simulink model "radia_optuna_teaching"  (R2026a)
settings: Solver=FixedStepDiscrete  StopTime=1.4  FixedStep=0.1
PreLoadFcn:
  | radia.simulink.makeOptunaMonitorBusObject();
model workspace (MAT data in the model file):
  radia_optuna_teaching_exercise = "quadratic"
  x = 0
settings Model: Creator=Administrator  LastModifiedBy=Administrator

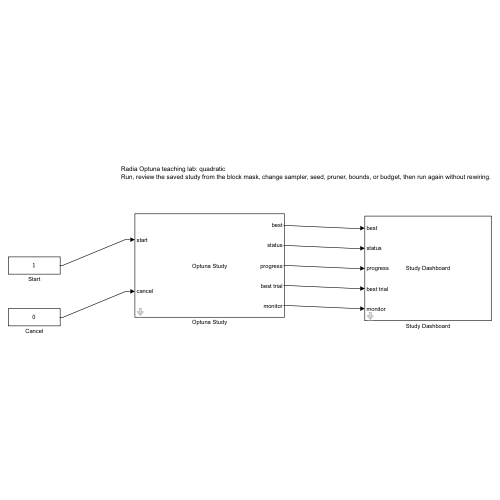
[thumbnail: Simulink's stored preview of the top-level diagram]
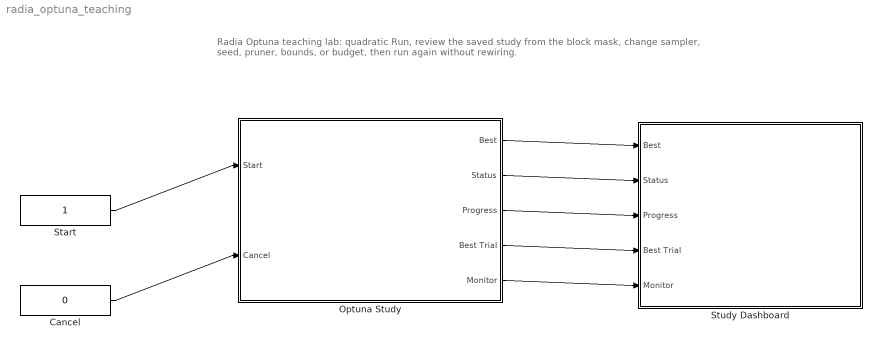
== system radia_optuna_teaching ==
  note: Radia Optuna teaching lab: quadratic
      | Run, review the saved study from the block mask, change sampler, seed, pruner, bounds, or budget, then run again without rewiring.
  Cancel : Constant  Value=0
  Optuna Study : Subsystem  mask{objective_fcn='radia.optuna.teachingQuadraticObjective', num_trials=12, directions="minimize", storage_path='C:\temp\radia_optuna_teaching_quadratic.mat', sample_time_s=0.10000000000000001, live_visualization=off, sampler_name=tpe, seed=20260829, pruner_name=median, parameter_spec=radia.optuna.OptimizationParameter('x',Value=0,Minimum=-1,Maximum=1), model_name='radia_optuna_teaching', selected_trial=-1}
      mask prompts: objective_fcn "Objective function"; num_trials "Total trial budget"; directions "Objective directions"; storage_path "Study MAT file"; sample_time_s "Trial sample time (s)"; live_visualization "External MATLAB monitor"; sampler_name "Sampler"; seed "Sampler seed ([] = fresh)"; pruner_name "Pruner"; parameter_spec "OptimizationParameter array"; model_name "Model to update"; selected_trial "Trial to apply (-1 = best)"
      mask help: Compact MATLAB-native Optuna study. Change the sampler, seed, pruner, search space, or total trial budget in this dialog and run again; the MAT study resumes without changing wiring. OptunaMonitorBusV1 exposes fixed scalar telemetry.
      mask init:
      | radia.simulink.makeOptunaMonitorBusObject();set_param([gcb '/Advanced Runtime'],'Parameters','objective_fcn,num_trials,directions,storage_path,sample_time_s,strcmp(live_visualization,''on''),struct(''Name'',sampler_name,''Seed'',seed,''Pruner'',pruner_name,''Parameters'',parameter_spec,''ModelName'',model_name)');
      mask TypeOptions sampler_name: auto | random | tpe | cmaes | motpe | nsgaii | gp | nsgaiii | bruteforce | qmc
      mask TypeOptions pruner_name: none | median | hyperband | percentile | patient | successivehalving | threshold
      mask DialogControl review_study Prompt: Review saved study
      mask DialogControl review_study Callback: radia.simulink.reviewOptunaStudy(gcb);
      mask DialogControl apply_trial Prompt: Apply selected trial
      mask DialogControl apply_trial Callback: radia.simulink.applyOptunaTrial(gcb,selected_trial);
      mask Display: disp('Optuna Study');port_label('input',1,'start');port_label('input',2,'cancel');port_label('output',1,'best');port_label('output',2,'status');port_label('output',3,'progress');port_label('output',4,'best trial');port_label('output',5,'monitor');
  Start : Constant
  Study Dashboard : Subsystem
      mask help: Compact live progress plus workspace logs. Full trial history remains in the Optuna Study MAT file.
      mask Display: disp('Study Dashboard');port_label('input',1,'best');port_label('input',2,'status');port_label('input',3,'progress');port_label('input',4,'best trial');port_label('input',5,'monitor');
  wires:
  Start/1 -> Optuna Study/1(Start)
  Cancel/1 -> Optuna Study/2(Cancel)
  Optuna Study/1(Best) -> Study Dashboard/1(Best)
  Optuna Study/2(Status) -> Study Dashboard/2(Status)
  Optuna Study/3(Progress) -> Study Dashboard/3(Progress)
  Optuna Study/4(Best Trial) -> Study Dashboard/4(Best Trial)
  Optuna Study/5(Monitor) -> Study Dashboard/5(Monitor)

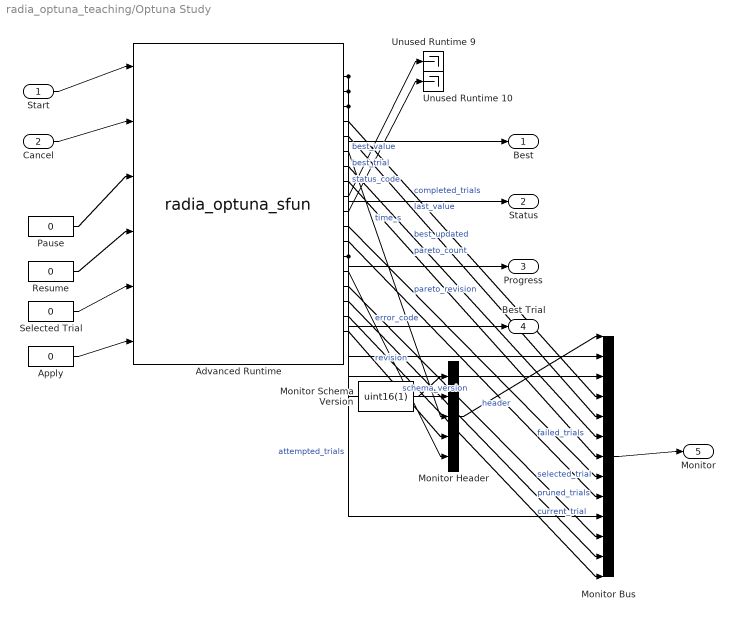
== system radia_optuna_teaching/Optuna Study ==
  Start : Inport
  Cancel : Inport  Port=2
  Advanced Runtime : M-S-Function  FunctionName=radia_optuna_sfun  Parameters=objective_fcn,num_trials,directions,storage_path,sample_time_s,strcmp(live_visualization,'on'),struct('Name',sampler_name,'Seed',seed,'Pruner',pruner_name,'Parameters',parameter_spec,'ModelName',model_name)
  Apply : Constant  Value=0
  Monitor Bus : BusCreator  Inputs=13  OutDataTypeStr=Bus: OptunaMonitorBusV1  NonVirtualBus=on
  Monitor Header : BusCreator  Inputs=5  OutDataTypeStr=Bus: RadiaMonitorHeaderV1  NonVirtualBus=on
  Monitor Schema Version : Constant  Value=uint16(1)  OutDataTypeStr=uint16
  Pause : Constant  Value=0
  Resume : Constant  Value=0
  Selected Trial : Constant  Value=0
  Unused Runtime 10 : Terminator
  Unused Runtime 9 : Terminator
  Best : Outport
  Status : Outport  Port=2
  Progress : Outport  Port=3
  Best Trial : Outport  Port=4
  Monitor : Outport  Port=5
  wires:
  Start/1 -> Advanced Runtime/1
  Cancel/1 -> Advanced Runtime/2
  Pause/1 -> Advanced Runtime/3
  Resume/1 -> Advanced Runtime/4
  Selected Trial/1 -> Advanced Runtime/5
  Apply/1 -> Advanced Runtime/6
  Advanced Runtime/1 -> Best/1, Monitor Bus/2  "best_value"
  Advanced Runtime/3 -> Status/1, Monitor Header/2  "status_code"
  Advanced Runtime/13 -> Progress/1, Monitor Bus/10  "attempted_trials"
  Advanced Runtime/2 -> Best Trial/1, Monitor Bus/3  "best_trial"
  Monitor Schema Version/1 -> Monitor Header/1  "schema_version"
  Advanced Runtime/6 -> Monitor Header/3  "time_s"
  Advanced Runtime/18 -> Monitor Header/4  "revision"
  Advanced Runtime/14 -> Monitor Header/5  "error_code"
  Monitor Header/1 -> Monitor Bus/1  "header"
  Advanced Runtime/4 -> Monitor Bus/4  "completed_trials"
  Advanced Runtime/5 -> Monitor Bus/5  "last_value"
  Advanced Runtime/7 -> Monitor Bus/6  "best_updated"
  Advanced Runtime/8 -> Monitor Bus/7  "pareto_count"
  Advanced Runtime/11 -> Monitor Bus/8  "pareto_revision"
  Advanced Runtime/12 -> Monitor Bus/9  "failed_trials"
  Advanced Runtime/15 -> Monitor Bus/11  "selected_trial"
  Advanced Runtime/16 -> Monitor Bus/12  "pruned_trials"
  Advanced Runtime/17 -> Monitor Bus/13  "current_trial"
  Monitor Bus/1 -> Monitor/1
  Advanced Runtime/9 -> Unused Runtime 9/1
  Advanced Runtime/10 -> Unused Runtime 10/1

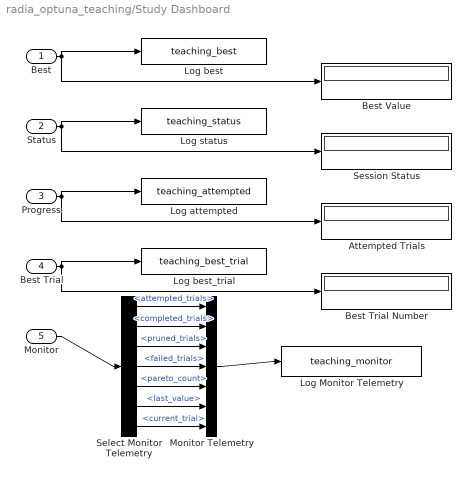
== system radia_optuna_teaching/Study Dashboard ==
  Best : Inport
  Status : Inport  Port=2
  Progress : Inport  Port=3
  Best Trial : Inport  Port=4
  Monitor : Inport  Port=5
  Attempted Trials : Display
  Best Trial Number : Display
  Best Value : Display
  Log Monitor Telemetry : ToWorkspace  VariableName=teaching_monitor  SampleTime=-1
  Log attempted : ToWorkspace  VariableName=teaching_attempted  SampleTime=-1
  Log best : ToWorkspace  VariableName=teaching_best  SampleTime=-1
  Log best_trial : ToWorkspace  VariableName=teaching_best_trial  SampleTime=-1
  Log status : ToWorkspace  VariableName=teaching_status  SampleTime=-1
  Monitor Telemetry : Mux  Inputs=7
  Select Monitor Telemetry : BusSelector  OutputSignals=attempted_trials,completed_trials,pruned_trials,failed_trials,pareto_count,last_value,current_trial
  Session Status : Display
  wires:
  Best/1 -> Log best/1, Best Value/1
  Status/1 -> Log status/1, Session Status/1
  Progress/1 -> Log attempted/1, Attempted Trials/1
  Best Trial/1 -> Log best_trial/1, Best Trial Number/1
  Monitor/1 -> Select Monitor Telemetry/1
  Select Monitor Telemetry/1 -> Monitor Telemetry/1  "<attempted_trials>"
  Select Monitor Telemetry/2 -> Monitor Telemetry/2  "<completed_trials>"
  Select Monitor Telemetry/3 -> Monitor Telemetry/3  "<pruned_trials>"
  Select Monitor Telemetry/4 -> Monitor Telemetry/4  "<failed_trials>"
  Select Monitor Telemetry/5 -> Monitor Telemetry/5  "<pareto_count>"
  Select Monitor Telemetry/6 -> Monitor Telemetry/6  "<last_value>"
  Select Monitor Telemetry/7 -> Monitor Telemetry/7  "<current_trial>"
  Monitor Telemetry/1 -> Log Monitor Telemetry/1
